simulink model "da"  (R2026a)
settings: Solver=VariableStepAuto  StopTime=720
settings Model: Creator=adhar  LastModifiedBy=adhar

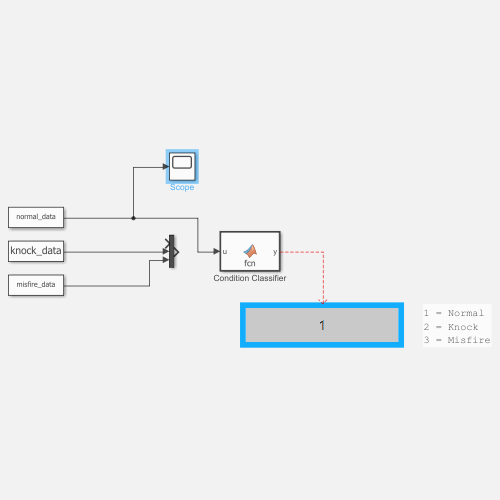
[thumbnail: Simulink's stored preview of the top-level diagram]
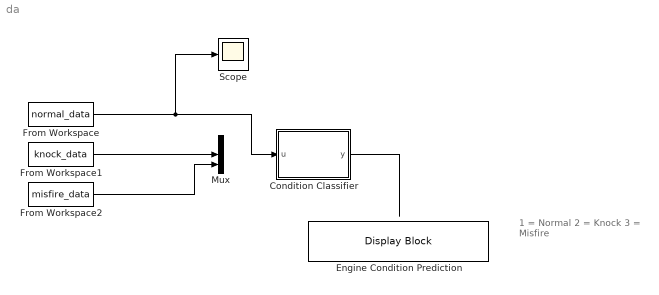
== system da ==
  note: 1 = Normal
      | 2 = Knock
      | 3 = Misfire
  Condition Classifier : MATLAB Function  TreatAsAtomicUnit=on
  Engine Condition Prediction : DisplayBlock  LabelPosition=Hide  Transparency=1  GridColor=[0.502, 0.502, 0.502]
  From Workspace : FromWorkspace  VariableName=normal_data  SampleTime=0.5
  From Workspace1 : FromWorkspace  VariableName=knock_data  SampleTime=0.5
  From Workspace2 : FromWorkspace  VariableName=misfire_data  SampleTime=0.5
  Mux : Mux  Inputs=3
  Scope : Scope
      settings: ActiveDisplayYMinimum=2.2204460492503131E-16
  wires:
  From Workspace/1 -> Scope/1, Condition Classifier/1(u)
  From Workspace1/1 -> Mux/2
  From Workspace2/1 -> Mux/3
  Condition Classifier/1(y) -> ?

== matlab function da/Condition Classifier ==
  data: u input; y output
function y = fcn(u)

persistent maxP

if isempty(maxP)
    maxP = u;
else
    maxP = max(maxP,u);
end

% Classify based on maximum cylinder pressure
if maxP < 4
    y = 3;          % Misfire
elseif maxP > 10
    y = 2;          % Knock
else
    y = 1;          % Normal
end
